simulink model "quarter_car_passive"  (R2025b)
settings: Solver=VariableStepAuto  StartTime=0.0  StopTime=10.0  RelTol=1e-3
settings Model: Creator=mvish  LastModifiedBy=mvish

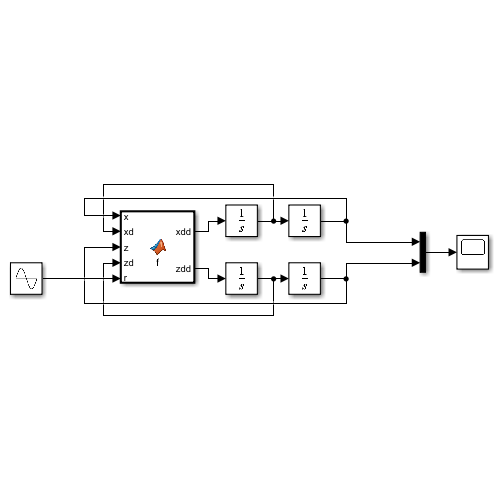
[thumbnail: Simulink's stored preview of the top-level diagram]
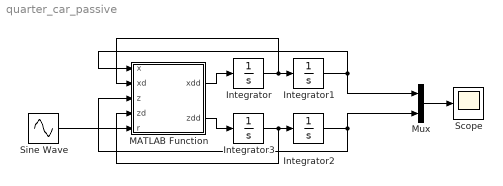
== system quarter_car_passive ==
  Integrator{,1..3} (4 alike) : Integrator
  MATLAB Function : MATLAB Function  TreatAsAtomicUnit=on
  Mux : Mux  Inputs=2
  Scope : Scope
      settings: ActiveDisplayYMinimum=-0.038178102723289926  ActiveDisplayYMaximum=0.038406826162738487
  Sine Wave : Sin  Amplitude=0.03  SampleTime=0
  wires:
  Integrator3/1 -> MATLAB Function/4(zd), Integrator2/1
  Integrator/1 -> MATLAB Function/2(xd), Integrator1/1
  MATLAB Function/1(xdd) -> Integrator/1
  MATLAB Function/2(zdd) -> Integrator3/1
  Sine Wave/1 -> MATLAB Function/5(r)
  Integrator1/1 -> Mux/1, MATLAB Function/1(x)
  Integrator2/1 -> MATLAB Function/3(z), Mux/2
  Mux/1 -> Scope/1

== matlab function quarter_car_passive/MATLAB Function ==
  data: x input; xdd output; xd input; z input; zd input; r input; zdd output
function [xdd,zdd] = f(x,xd,z,zd,r)

ms = 250;
mu = 40;
k  = 16000;
b  = 1000;
kt = 190000;


xdd = (-b*(xd-zd) - k*(x-z))/ms;

zdd = ( b*(xd-zd) + k*(x-z) - kt*(z-r))/mu;

end
